simulink model "ex3"  (R2025b)
settings: Solver=FixedStepAuto  StartTime=0.0  StopTime=0.35  FixedStep=1e-5  RelTol=1e-4
values from neighbouring files (symbols this model uses):
  ba = (as*J-b)/psi    [sim1.m]
  In = 20    [sim1.m]
  J = 0.001    [sim1.m]
  ki = ac^2*L    [sim1.m]
  kis = bn*as/psi    [sim1.m]
  kp = ac*L    [sim1.m]
  kps = as*J/psi    [sim1.m]
  L = 2.5e-3    (= 0.0025)    [sim1.m]
  psi = 0.35    [sim1.m]
  R = 0.5    [sim1.m]
  Ra = ac*L-R    [sim1.m]
  Tn = 7    [sim1.m]
  Vn = 120    [sim1.m]
  wn = Nn*2*pi/60    (= 314.159265359)    [sim1.m]
settings Model: Creator=dimit  LastModifiedBy=Dimitris

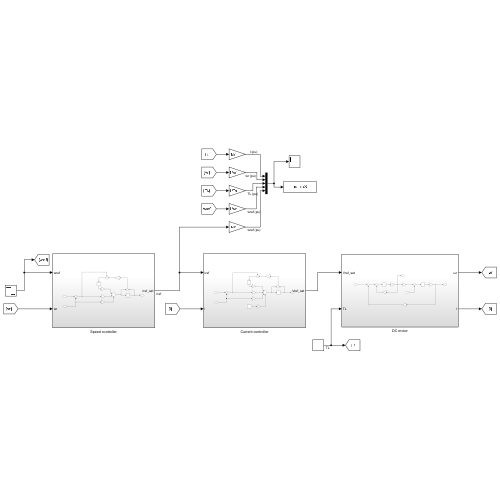
[thumbnail: Simulink's stored preview of the top-level diagram]
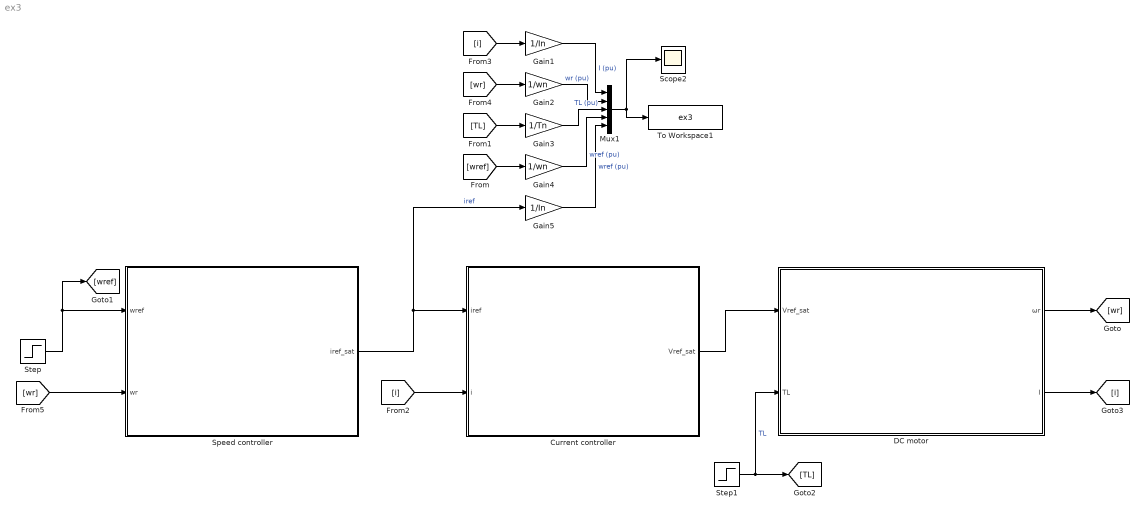
== system ex3 ==
  Current controller : Subsystem
  DC motor : Subsystem
  Gain1 : Gain  Gain=1/In
  Gain2 : Gain  Gain=1/wn
  Gain3 : Gain  Gain=1/Tn
  Gain4 : Gain  Gain=1/wn
  Gain5 : Gain  Gain=1/In
  Mux1 : Mux  Inputs=5
  Scope2 : Scope
      settings: ActiveDisplayYMinimum=-7.0867458110982913  ActiveDisplayYMaximum=12.069160745283463  DataLoggingVariableName=ScopeData2
  Speed controller : Subsystem
  Step : Step  Time=0.07  Before=wn  After=wn-160  SampleTime=0
  Step1 : Step  Time=0.15  After=Tn  SampleTime=0
  To Workspace1 : ToWorkspace  VariableName=ex3  SaveFormat=Timeseries  SampleTime=-1
  wires:
  Current controller/1(Vref_sat) -> DC motor/1(Vref_sat)
  Speed controller/1(iref_sat) -> Gain5/1, Current controller/1(iref)  "iref"
  [i] -> Current controller/2(i)
  DC motor/1(ωr) -> [wr]
  Step/1 -> Speed controller/1(wref), [wref]
  [i] -> Gain1/1
  Mux1/1 -> To Workspace1/1, Scope2/1
  Gain2/1 -> Mux1/2  "wr (pu)"
  Gain1/1 -> Mux1/1  "I (pu)"
  [wr] -> Gain2/1
  [TL] -> Gain3/1
  [wref] -> Gain4/1
  Gain3/1 -> Mux1/3  "TL (pu)"
  Gain4/1 -> Mux1/4  "wref (pu)"
  Step1/1 -> [TL], DC motor/2(TL)  "TL"
  Gain5/1 -> Mux1/5  "wref (pu)"
  DC motor/2(I) -> [i]
  [wr] -> Speed controller/2(wr)

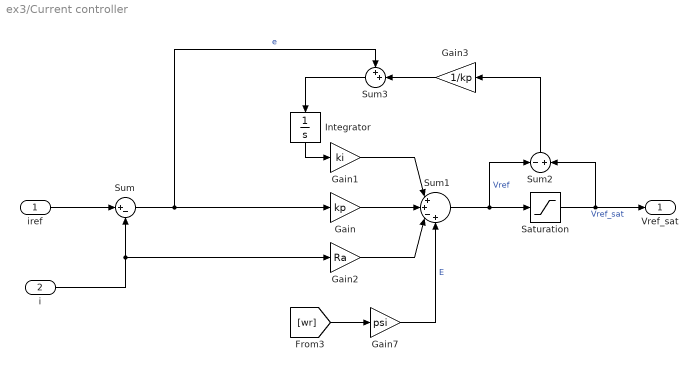
== system ex3/Current controller ==
  iref : Inport
  i : Inport  Port=2
  Gain : Gain  Gain=kp
  Gain1 : Gain  Gain=ki
  Gain2 : Gain  Gain=Ra
  Gain3 : Gain  Gain=1/kp
  Gain7 : Gain  Gain=psi
  Integrator : Integrator
  Saturation : Saturate  UpperLimit=Vn  LowerLimit=-Vn
  Sum : Sum  Inputs=|+-
  Sum1 : Sum  Inputs=|++-+
  Sum2 : Sum  Inputs=-|+
  Sum3 : Sum  Inputs=++|
  Vref_sat : Outport
  wires:
  Saturation/1 -> Vref_sat/1, Sum2/2  "Vref_sat"
  Sum2/1 -> Gain3/1
  Sum3/1 -> Integrator/1
  Gain7/1 -> Sum1/4  "E"
  [wr] -> Gain7/1
  Gain3/1 -> Sum3/2
  Sum1/1 -> Sum2/1, Saturation/1  "Vref"
  Gain/1 -> Sum1/2
  i/1 -> Sum/2, Gain2/1
  Sum/1 -> Sum3/1, Gain/1  "e"
  Gain2/1 -> Sum1/3
  Gain1/1 -> Sum1/1
  iref/1 -> Sum/1
  Integrator/1 -> Gain1/1

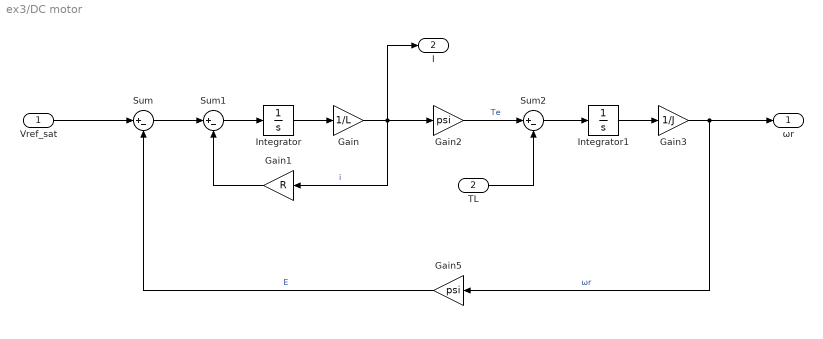
== system ex3/DC motor ==
  Vref_sat : Inport
  TL : Inport  Port=2
  Gain : Gain  Gain=1/L
  Gain1 : Gain  Gain=R
  Gain2 : Gain  Gain=psi
  Gain3 : Gain  Gain=1/J
  Gain5 : Gain  Gain=psi
  Integrator : Integrator
  Integrator1 : Integrator
  Sum : Sum  Inputs=|+-
  Sum1 : Sum  Inputs=|+-
  Sum2 : Sum  Inputs=|+-
  ωr : Outport
  I : Outport  Port=2
  wires:
  Gain/1 -> Gain1/1, I/1, Gain2/1  "i"
  Gain2/1 -> Sum2/1  "Te"
  Sum/1 -> Sum1/1
  Integrator1/1 -> Gain3/1
  Integrator/1 -> Gain/1
  Gain3/1 -> ωr/1, Gain5/1  "ωr"
  Sum2/1 -> Integrator1/1
  Gain5/1 -> Sum/2  "E"
  Gain1/1 -> Sum1/2
  Sum1/1 -> Integrator/1
  Vref_sat/1 -> Sum/1
  TL/1 -> Sum2/2

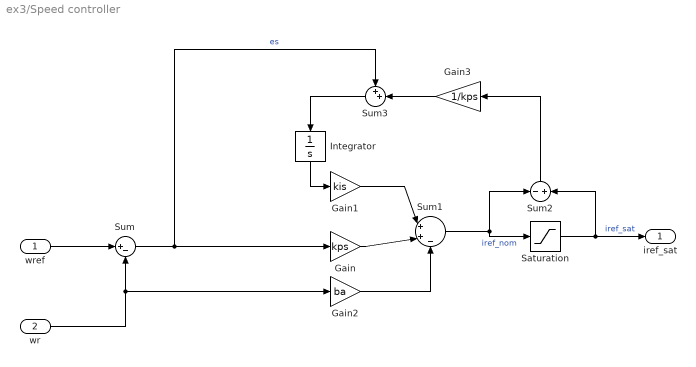
== system ex3/Speed controller ==
  wref : Inport
  wr : Inport  Port=2
  Gain : Gain  Gain=kps
  Gain1 : Gain  Gain=kis
  Gain2 : Gain  Gain=ba
  Gain3 : Gain  Gain=1/kps
  Integrator : Integrator
  Saturation : Saturate  UpperLimit=In*3  LowerLimit=-In*3
  Sum : Sum  Inputs=|+-
  Sum1 : Sum  Inputs=|++-
  Sum2 : Sum  Inputs=-|+
  Sum3 : Sum  Inputs=++|
  iref_sat : Outport
  wires:
  Saturation/1 -> iref_sat/1, Sum2/2  "iref_sat"
  Sum2/1 -> Gain3/1
  Gain3/1 -> Sum3/2
  Sum1/1 -> Saturation/1, Sum2/1  "iref_nom"
  Gain/1 -> Sum1/2
  wr/1 -> Sum/2, Gain2/1
  Sum/1 -> Sum3/1, Gain/1  "es"
  Gain2/1 -> Sum1/3
  Gain1/1 -> Sum1/1
  wref/1 -> Sum/1
  Integrator/1 -> Gain1/1
  Sum3/1 -> Integrator/1
